simulink model "quadratura"  (Simulink 7.7)
settings: Solver=ode45  StartTime=0.0  StopTime=10.0  MaxStep=1e-2  MinStep=1e-3  RelTol=1e-3
settings Model: Creator=vparro  LastModifiedBy=vanderleiparro
settings DebuggingCC: StrictBusMsg=Warning

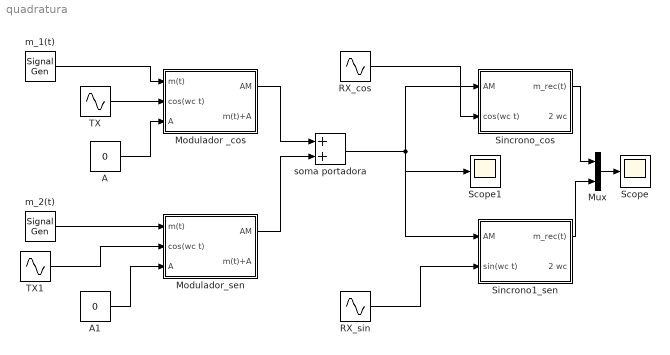
== system quadratura ==
  A : Constant  Value=0
  A1 : Constant  Value=0
  Modulador _cos : Subsystem
  Modulador_sen : Subsystem
  Mux : Mux  Inputs=2
  RX_cos : Sin  Frequency=20*pi  SampleTime=0
  RX_sin : Sin  Frequency=20*pi  Phase=-pi/2  SampleTime=0
  Scope : Scope
  Scope1 : Scope
  Sincrono1_sen : Subsystem
  Sincrono_cos : Subsystem
  TX : Sin  Frequency=20*pi  SampleTime=0
  TX1 : Sin  Frequency=20*pi  Phase=-pi/2  SampleTime=0
  m_1(t) : SignalGenerator  Frequency=1/5
  m_2(t) : SignalGenerator  Frequency=1/10
  soma portadora : Sum
  wires:
  TX/1 -> Modulador _cos/2(cos(wc t))
  m_1(t)/1 -> Modulador _cos/1(m(t))
  A/1 -> Modulador _cos/3(A)
  A1/1 -> Modulador_sen/3(A)
  TX1/1 -> Modulador_sen/2(cos(wc t))
  m_2(t)/1 -> Modulador_sen/1(m(t))
  Modulador _cos/1(AM) -> soma portadora/1
  Modulador_sen/1(AM) -> soma portadora/2
  soma portadora/1 -> Sincrono_cos/1(AM), Sincrono1_sen/1(AM), Scope1/1
  RX_sin/1 -> Sincrono1_sen/2(sin(wc t))
  RX_cos/1 -> Sincrono_cos/2(cos(wc t))
  Mux/1 -> Scope/1
  Sincrono_cos/1(m_rec(t)) -> Mux/1
  Sincrono1_sen/1(m_rec(t)) -> Mux/2

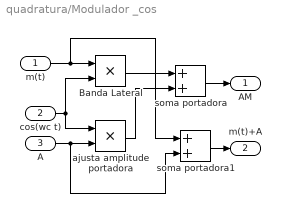
== system quadratura/Modulador _cos ==
  m(t) : Inport
  cos(wc t) : Inport  Port=2
  A : Inport  Port=3
  Banda Lateral : Product  RndMeth=Zero
  ajusta amplitude portadora : Product  RndMeth=Zero
  soma portadora : Sum
  soma portadora1 : Sum
  AM : Outport
  m(t)+A : Outport  Port=2
  wires:
  Banda Lateral/1 -> soma portadora/1
  soma portadora/1 -> AM/1
  cos(wc t)/1 -> ajusta amplitude portadora/1, Banda Lateral/2
  ajusta amplitude portadora/1 -> soma portadora/2
  A/1 -> soma portadora1/2, ajusta amplitude portadora/2
  m(t)/1 -> soma portadora1/1, Banda Lateral/1
  soma portadora1/1 -> m(t)+A/1

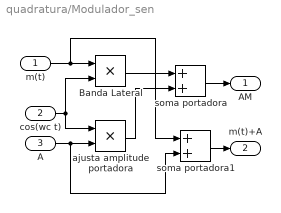
== system quadratura/Modulador_sen ==
  m(t) : Inport
  cos(wc t) : Inport  Port=2
  A : Inport  Port=3
  Banda Lateral : Product  RndMeth=Zero
  ajusta amplitude portadora : Product  RndMeth=Zero
  soma portadora : Sum
  soma portadora1 : Sum
  AM : Outport
  m(t)+A : Outport  Port=2
  wires:
  soma portadora1/1 -> m(t)+A/1
  m(t)/1 -> Banda Lateral/1, soma portadora1/1
  A/1 -> ajusta amplitude portadora/2, soma portadora1/2
  ajusta amplitude portadora/1 -> soma portadora/2
  cos(wc t)/1 -> Banda Lateral/2, ajusta amplitude portadora/1
  soma portadora/1 -> AM/1
  Banda Lateral/1 -> soma portadora/1

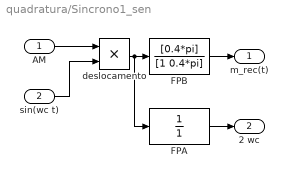
== system quadratura/Sincrono1_sen ==
  AM : Inport
  sin(wc t) : Inport  Port=2
  FPA : TransferFcn  Denominator=[1]
  FPB : TransferFcn  Numerator=[0.4*pi]  Denominator=[1 0.4*pi]
  deslocamento : Product  RndMeth=Zero
  m_rec(t) : Outport
  2 wc : Outport  Port=2
  wires:
  FPA/1 -> 2 wc/1
  FPB/1 -> m_rec(t)/1
  deslocamento/1 -> FPA/1, FPB/1
  sin(wc t)/1 -> deslocamento/2
  AM/1 -> deslocamento/1

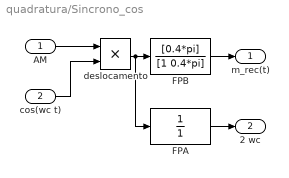
== system quadratura/Sincrono_cos ==
  AM : Inport
  cos(wc t) : Inport  Port=2
  FPA : TransferFcn  Denominator=[1]
  FPB : TransferFcn  Numerator=[0.4*pi]  Denominator=[1 0.4*pi]
  deslocamento : Product  RndMeth=Zero
  m_rec(t) : Outport
  2 wc : Outport  Port=2
  wires:
  AM/1 -> deslocamento/1
  cos(wc t)/1 -> deslocamento/2
  deslocamento/1 -> FPB/1, FPA/1
  FPB/1 -> m_rec(t)/1
  FPA/1 -> 2 wc/1
